simulink model "Ejercicio_4_2"  (R2026b)
settings: Solver=VariableStepAuto  StopTime=t_stop
InitFcn:
  | caso_run = '4.2'; pv_params; clear caso_run
values from neighbouring files (symbols this model uses):
  alpha0 = fzero(f, [0 1])    [pv_params(1).m]    (also in pv_params(2).m; pv_params(3).m; pv_params(4).m; pv_params.m)
  comedelay = 20e-3    (= 0.02)    [pv_params(1).m]    (also in pv_params(2).m; pv_params(3).m; pv_params(4).m; pv_params.m)
  Pinv_nom = 2000    [pv_params(1).m]    (also in pv_params(2).m; pv_params(3).m; pv_params(4).m; pv_params.m)
  Ppcc0 = sum(min(alpha0*Pinv_nom, Pavail))    [pv_params(1).m]    (also in pv_params(2).m; pv_params(3).m; pv_params(4).m; pv_params.m)
  t_sample_ppc = 0.2    [pv_params(1).m]    (also in pv_params(2).m; pv_params(3).m; pv_params(4).m; pv_params.m)
  tau_pv = 0.5    [pv_params(1).m]    (also in pv_params(2).m; pv_params(3).m; pv_params(4).m; pv_params.m)
libraries: sl_discontinuities x5
settings Model: Creator=mithu  LastModifiedBy=mithu

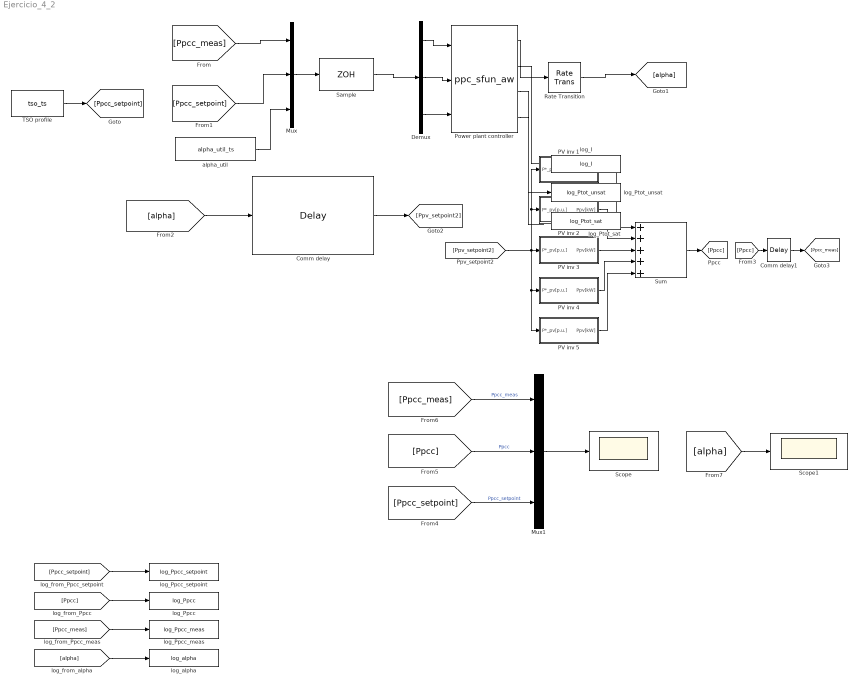
== system Ejercicio_4_2 ==
  Comm delay : TransportDelay  DelayTime=comedelay  InitialOutput=alpha0
  Comm delay1 : TransportDelay  DelayTime=comedelay  InitialOutput=Ppcc0
  Demux : Demux  Outputs=3
  Mux : Mux  Inputs=3
  Mux1 : Mux  Inputs=3
  PV inv 1 : Subsystem
  PV inv 2 : Subsystem
  PV inv 3 : Subsystem
  PV inv 4 : Subsystem
  PV inv 5 : Subsystem
  Power plant controller : M-S-Function  FunctionName=ppc_sfun_aw  Parameters=t_sample_ppc, Kp, Ki, Ppv_nom, ppc_mode, I0, aw_mode
  Rate Transition : RateTransition  Integrity=off  InitialCondition=alpha0
  Sample : ZeroOrderHold  SampleTime=t_sample_ppc
  Scope : Scope
      settings: ActiveDisplayYMinimum=4375  ActiveDisplayYMaximum=10625.000000000004
  Scope1 : Scope
      settings: ActiveDisplayYMinimum=0.4375  ActiveDisplayYMaximum=1.0625
  Sum : Sum  Inputs=+++++
  TSO profile : FromWorkspace  VariableName=tso_ts  Interpolate=off  OutputAfterFinalValue=Holding final value
  alpha_util : FromWorkspace  VariableName=alpha_util_ts  Interpolate=off  OutputAfterFinalValue=Holding final value
  log_I : ToWorkspace  VariableName=log_I  SaveFormat=Timeseries  SampleTime=-1
  log_Ppcc : ToWorkspace  VariableName=log_Ppcc  SaveFormat=Timeseries  SampleTime=-1
  log_Ppcc_meas : ToWorkspace  VariableName=log_Ppcc_meas  SaveFormat=Timeseries  SampleTime=-1
  log_Ppcc_setpoint : ToWorkspace  VariableName=log_Ppcc_setpoint  SaveFormat=Timeseries  SampleTime=-1
  log_Ptot_sat : ToWorkspace  VariableName=log_Ptot_sat  SaveFormat=Timeseries  SampleTime=-1
  log_Ptot_unsat : ToWorkspace  VariableName=log_Ptot_unsat  SaveFormat=Timeseries  SampleTime=-1
  log_alpha : ToWorkspace  VariableName=log_alpha  SaveFormat=Timeseries  SampleTime=-1
  wires:
  [Ppcc_meas] -> Mux/1
  [Ppcc_setpoint] -> Mux/2
  Mux/1 -> Sample/1
  Sample/1 -> Demux/1
  Demux/1 -> Power plant controller/1
  Demux/2 -> Power plant controller/2
  Power plant controller/1 -> Rate Transition/1
  Rate Transition/1 -> [alpha]
  [alpha] -> Comm delay/1
  Comm delay/1 -> [Ppv_setpoint2]
  [Ppv_setpoint2] -> PV inv 1/1(P*_pv[p.u.]), PV inv 2/1(P*_pv[p.u.]), PV inv 5/1(P*_pv[p.u.]), PV inv 4/1(P*_pv[p.u.]), PV inv 3/1(P*_pv[p.u.])
  PV inv 1/1(Ppv[kW]) -> Sum/1
  PV inv 3/1(Ppv[kW]) -> Sum/3
  PV inv 4/1(Ppv[kW]) -> Sum/4
  PV inv 5/1(Ppv[kW]) -> Sum/5
  PV inv 2/1(Ppv[kW]) -> Sum/2
  Sum/1 -> [Ppcc]
  [Ppcc] -> Comm delay1/1
  Comm delay1/1 -> [Ppcc_meas]
  [Ppcc_meas] -> Mux1/1  "Ppcc_meas"
  [Ppcc] -> Mux1/2  "Ppcc"
  [Ppcc_setpoint] -> Mux1/3  "Ppcc_setpoint"
  Mux1/1 -> Scope/1
  [alpha] -> Scope1/1
  [Ppcc_setpoint] -> log_Ppcc_setpoint/1
  [Ppcc] -> log_Ppcc/1
  [Ppcc_meas] -> log_Ppcc_meas/1
  [alpha] -> log_alpha/1
  TSO profile/1 -> [Ppcc_setpoint]
  alpha_util/1 -> Mux/3
  Demux/3 -> Power plant controller/3
  Power plant controller/2 -> log_I/1
  Power plant controller/3 -> log_Ptot_unsat/1
  Power plant controller/4 -> log_Ptot_sat/1

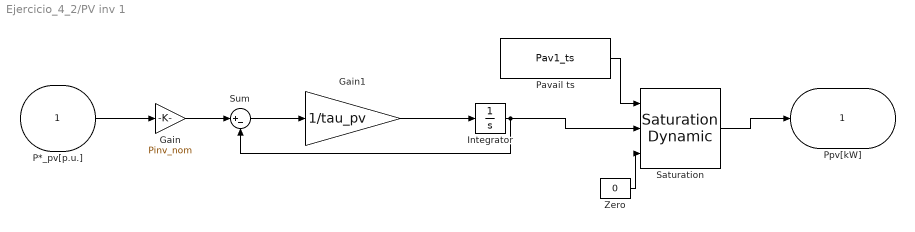
== system Ejercicio_4_2/PV inv 1 ==
  P*_pv[p.u.] : Inport
  Gain : Gain  Gain=Pinv_nom
  Gain1 : Gain  Gain=1/tau_pv
  Integrator : Integrator  InitialCondition=alpha0*Pinv_nom
  Pavail ts : FromWorkspace  VariableName=Pav1_ts  Interpolate=off  OutputAfterFinalValue=Holding final value
  Saturation : sl_discontinuities/Saturation Dynamic  OutMin=[]  OutMax=[]  OutDataTypeStr=Inherit: Same as second input  OutDataType=fixdt(1, 16)  OutScaling=2^-10  DoSatur=off
      settings: LibrarySourceBlock=|
      | simulink/Discontinuities/Saturation
      | Dynamic
  Sum : Sum  Inputs=|+-
  Zero : Constant  Value=0
  Ppv[kW] : Outport
  wires:
  P*_pv[p.u.]/1 -> Gain/1
  Gain/1 -> Sum/1
  Sum/1 -> Gain1/1
  Gain1/1 -> Integrator/1
  Integrator/1 -> Saturation/2, Sum/2
  Pavail ts/1 -> Saturation/1
  Zero/1 -> Saturation/3
  Saturation/1 -> Ppv[kW]/1

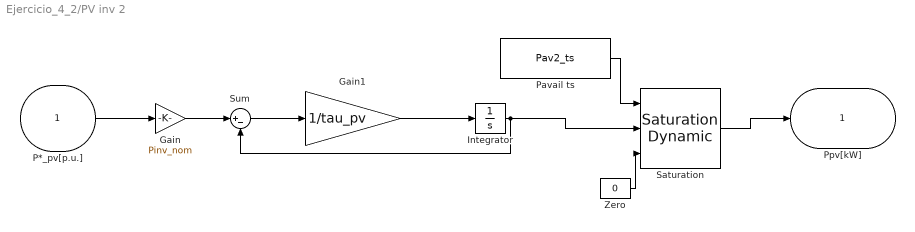
== system Ejercicio_4_2/PV inv 2 ==
  P*_pv[p.u.] : Inport
  Gain : Gain  Gain=Pinv_nom
  Gain1 : Gain  Gain=1/tau_pv
  Integrator : Integrator  InitialCondition=alpha0*Pinv_nom
  Pavail ts : FromWorkspace  VariableName=Pav2_ts  Interpolate=off  OutputAfterFinalValue=Holding final value
  Saturation : sl_discontinuities/Saturation Dynamic  OutMin=[]  OutMax=[]  OutDataTypeStr=Inherit: Same as second input  OutDataType=fixdt(1, 16)  OutScaling=2^-10  DoSatur=off
      settings: LibrarySourceBlock=|
      | simulink/Discontinuities/Saturation
      | Dynamic
  Sum : Sum  Inputs=|+-
  Zero : Constant  Value=0
  Ppv[kW] : Outport
  wires:
  P*_pv[p.u.]/1 -> Gain/1
  Gain/1 -> Sum/1
  Sum/1 -> Gain1/1
  Gain1/1 -> Integrator/1
  Integrator/1 -> Saturation/2, Sum/2
  Pavail ts/1 -> Saturation/1
  Zero/1 -> Saturation/3
  Saturation/1 -> Ppv[kW]/1

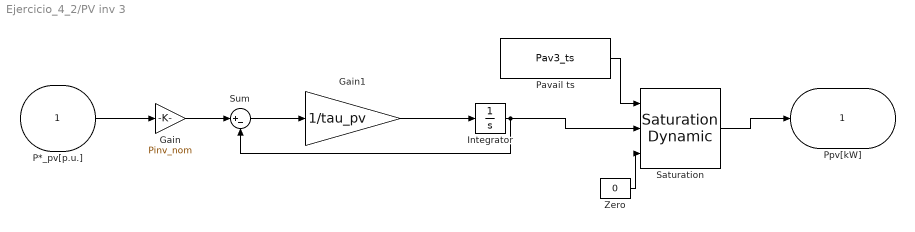
== system Ejercicio_4_2/PV inv 3 ==
  P*_pv[p.u.] : Inport
  Gain : Gain  Gain=Pinv_nom
  Gain1 : Gain  Gain=1/tau_pv
  Integrator : Integrator  InitialCondition=alpha0*Pinv_nom
  Pavail ts : FromWorkspace  VariableName=Pav3_ts  Interpolate=off  OutputAfterFinalValue=Holding final value
  Saturation : sl_discontinuities/Saturation Dynamic  OutMin=[]  OutMax=[]  OutDataTypeStr=Inherit: Same as second input  OutDataType=fixdt(1, 16)  OutScaling=2^-10  DoSatur=off
      settings: LibrarySourceBlock=|
      | simulink/Discontinuities/Saturation
      | Dynamic
  Sum : Sum  Inputs=|+-
  Zero : Constant  Value=0
  Ppv[kW] : Outport
  wires:
  P*_pv[p.u.]/1 -> Gain/1
  Gain/1 -> Sum/1
  Sum/1 -> Gain1/1
  Gain1/1 -> Integrator/1
  Integrator/1 -> Saturation/2, Sum/2
  Pavail ts/1 -> Saturation/1
  Zero/1 -> Saturation/3
  Saturation/1 -> Ppv[kW]/1

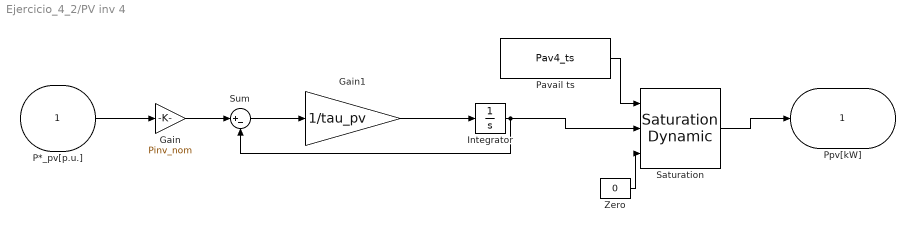
== system Ejercicio_4_2/PV inv 4 ==
  P*_pv[p.u.] : Inport
  Gain : Gain  Gain=Pinv_nom
  Gain1 : Gain  Gain=1/tau_pv
  Integrator : Integrator  InitialCondition=alpha0*Pinv_nom
  Pavail ts : FromWorkspace  VariableName=Pav4_ts  Interpolate=off  OutputAfterFinalValue=Holding final value
  Saturation : sl_discontinuities/Saturation Dynamic  OutMin=[]  OutMax=[]  OutDataTypeStr=Inherit: Same as second input  OutDataType=fixdt(1, 16)  OutScaling=2^-10  DoSatur=off
      settings: LibrarySourceBlock=|
      | simulink/Discontinuities/Saturation
      | Dynamic
  Sum : Sum  Inputs=|+-
  Zero : Constant  Value=0
  Ppv[kW] : Outport
  wires:
  P*_pv[p.u.]/1 -> Gain/1
  Gain/1 -> Sum/1
  Sum/1 -> Gain1/1
  Gain1/1 -> Integrator/1
  Integrator/1 -> Saturation/2, Sum/2
  Pavail ts/1 -> Saturation/1
  Zero/1 -> Saturation/3
  Saturation/1 -> Ppv[kW]/1

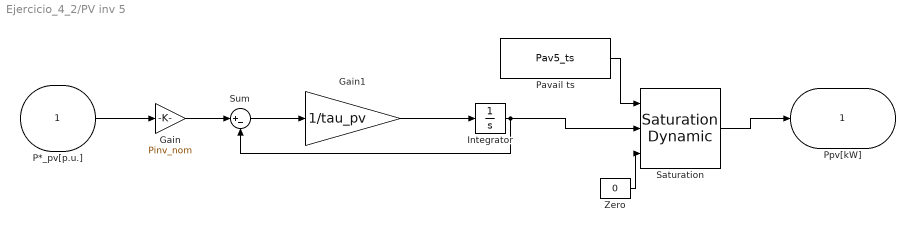
== system Ejercicio_4_2/PV inv 5 ==
  P*_pv[p.u.] : Inport
  Gain : Gain  Gain=Pinv_nom
  Gain1 : Gain  Gain=1/tau_pv
  Integrator : Integrator  InitialCondition=alpha0*Pinv_nom
  Pavail ts : FromWorkspace  VariableName=Pav5_ts  Interpolate=off  OutputAfterFinalValue=Holding final value
  Saturation : sl_discontinuities/Saturation Dynamic  OutMin=[]  OutMax=[]  OutDataTypeStr=Inherit: Same as second input  OutDataType=fixdt(1, 16)  OutScaling=2^-10  DoSatur=off
      settings: LibrarySourceBlock=|
      | simulink/Discontinuities/Saturation
      | Dynamic
  Sum : Sum  Inputs=|+-
  Zero : Constant  Value=0
  Ppv[kW] : Outport
  wires:
  P*_pv[p.u.]/1 -> Gain/1
  Gain/1 -> Sum/1
  Sum/1 -> Gain1/1
  Gain1/1 -> Integrator/1
  Integrator/1 -> Saturation/2, Sum/2
  Pavail ts/1 -> Saturation/1
  Zero/1 -> Saturation/3
  Saturation/1 -> Ppv[kW]/1
